simulink model "ChoiSul1996_DeadTime"  (R2024b)
settings: Solver=FixedStepDiscrete  StartTime=0.0  StopTime=Duration  FixedStep=h  RelTol=1e-3
InitFcn:
  | demoModel=bdroot; demoWorkspace=get_param(demoModel,'ModelWorkspace');
  | demoCases=getVariable(demoWorkspace,'DemoCases');
  | demoCaseName=get_param([demoModel '/Experiment_Settings'],'CaseName');
  | demoSelected=find(strcmp(demoCaseName,{demoCases.name}),1);
  | demoValues=demoCases(demoSelected).variables; demoNames=fieldnames(demoValues);
  | for demoIndex=1:numel(demoNames), assignin(demoWorkspace,demoNames{demoIndex},demoValues.(demoNames{demoIndex})); end
  | clear demoModel demoWorkspace demoCases demoCaseName demoSelected demoValues demoNames demoIndex;
model workspace (MAT data in the model file):
  CompDuty = 0.0266762524843
  DemoCases(1).name = 'No_compensation'
  DemoCases(1).variables.CompDuty = 0
  DemoCases(1).variables.UseWeakening = 0
  DemoCases(2).name = 'Calibrated_compensation'
  DemoCases(2).variables.CompDuty = 0.0266762524843
  DemoCases(2).variables.UseWeakening = 0
  SpeedProgram = [0  0; 0.12  300; 0.9  300]
  UseWeakening = 0
values from neighbouring files (symbols this model uses):
  B = 0.0002    [ChoiSul1996_DeadTime.sldd]
  BaseCap = 11.4197598 11.4197598 11.4197598 11.4197598 11.4197598 11.4197598 11.4197598 11.4197598 11.4197598 11.4197598 11.4197598 11.4197598 11.4197598 11.4197598 11.4197598 11.4197598 11.4197598 11.4197598 11.4197598 11.4197598 11.4197598 11.4197598 11.4197598 11.4197598 11.4197598 11.4197598 11.4197598 11.4197598 11.4197598 11.4197598 11.4197598 11.4197598 11.4197598 11.4197598 11.4197598 11.4197598 11.4    [ChoiSul1996_DeadTime.sldd]
  BaseId = -0.0 -0.0 -0.0 -0.0 -0.0 -0.0 -0.0 -0.0 -0.0 -0.0 -0.0 -0.0 -0.0 -0.0 -0.0 -0.0 -0.0 -0.0 -0.0 -0.0 -0.0 -0.0 -0.0 -0.0 -0.0 -0.0 -0.0 -0.0 -0.0 -0.0 -0.0 -0.0 -0.0 -0.0 -0.0 -0.0 -0.0 -0.0 -0.0 -0.0 -0.0 -0.0 -0.0 -0.0 -0.0 -0.0 -0.0 -0.0 -0.0 -0.0 -0.0 -0.0 -0.0 -0.0 -0.0 -0.0 -0.0 -0.0 -0.0 -0.0 -0.0 -0.0 -0.0 -0.0 -0.0 -0.0 -0.0 -0.0 -0.0 -0.0 -0.0 -0.0 -0.0 -0.0 -0.0 -0.0 -0.0 -0.0 -0.0 -0.0    [ChoiSul1996_DeadTime.sldd]
  BaseIq = 0.0 0.0 0.0 0.0 0.0 0.0 0.0 0.0 0.0 0.0 0.0 0.0 0.0 0.0 0.0 0.0 0.0 0.0 0.0 0.0 0.0 0.0 0.0 0.0 0.0 0.0 0.0 0.0 0.0 0.0 0.0 0.0 0.0 0.0 0.0 0.0 0.0 0.0 0.0 0.0 0.0 0.0 0.0 0.0 0.0 0.0 0.0 0.0 0.0 0.0 0.0 0.0 0.0 0.0 0.0 0.0 0.0 0.0 0.0 0.0 0.0 0.0 0.0 0.0 0.0 0.0 0.0 0.0 0.0 0.0 0.0 0.0 0.0 0.0 0.0 0.0 0.0 0.0 0.0 0.0 0.0 0.0 0.0 0.0 0.0 0.0 0.0 0.0 0.0 0.0 0.0 0.0 0.0 0.0 0.0 0.0 0.0 0.0 0.0 0.0    [ChoiSul1996_DeadTime.sldd]
  BusReadyRatio = 0.94    [ChoiSul1996_DeadTime.sldd]
  CurrentBandwidth = 1450.0    [ChoiSul1996_DeadTime.sldd]
  CurrentKaw = 1500.0    [ChoiSul1996_DeadTime.sldd]
  EdgePredict = 0.27    [ChoiSul1996_DeadTime.sldd]
  EnableThreshold = 0.5    [ChoiSul1996_DeadTime.sldd]
  Fraction = 0.0 0.025 0.05 0.075 0.1 0.125 0.15 0.175 0.2 0.225 0.25 0.275 0.3 0.325 0.35 0.375 0.4 0.425 0.45 0.475 0.5 0.525 0.55 0.575 0.6 0.625 0.65 0.675 0.7 0.725 0.75 0.775 0.8 0.825 0.85 0.875 0.9 0.925 0.95 0.975 1.0    [ChoiSul1996_DeadTime.sldd]
  FwCap = 11.4197598 11.4197598 11.4197598 11.4197598 11.4197598 11.4197598 11.4197598 11.4197598 11.4197598 11.4197598 11.4197598 11.4197598 11.4197598 11.4197598 11.4197598 11.4197598 11.4197598 11.4197598 11.4197598 11.4197598 11.4197598 11.4197598 11.4197598 11.4197598 11.4197598 11.4197598 11.4197598 11.4197598 11.4197598 11.4197598 11.4197598 11.4197598 11.4197598 11.4197598 11.4197598 11.4197598 11.4    [ChoiSul1996_DeadTime.sldd]
  FwId = -0.0 -0.0 -0.0 -0.0 -0.0 -0.0 -0.0 -0.0 -0.0 -0.0 -0.0 -0.0 -0.0 -0.0 -0.0 -0.0 -0.0 -0.0 -0.0 -0.0 -0.0 -0.0 -0.0 -0.0 -0.0 -0.0 -0.0 -0.0 -0.0 -0.0 -0.0 -0.0 -0.0 -0.0 -0.0 -0.0 -0.0 -0.0 -0.0 -0.0 -0.0 -0.0 -0.0 -0.0 -0.0 -0.0 -0.0 -0.0 -0.0 -0.0 -0.0 -0.0 -0.0 -0.0 -0.0 -0.0 -0.0 -0.0 -0.0 -0.0 -0.0 -0.0 -0.0 -0.0 -0.0 -0.0 -0.0 -0.0 -0.0 -0.0 -0.0 -0.0 -0.0 -0.0 -0.0 -0.0 -0.0 -0.0 -0.0 -0.0    [ChoiSul1996_DeadTime.sldd]
  FwIq = 0.0 0.0 0.0 0.0 0.0 0.0 0.0 0.0 0.0 0.0 0.0 0.0 0.0 0.0 0.0 0.0 0.0 0.0 0.0 0.0 0.0 0.0 0.0 0.0 0.0 0.0 0.0 0.0 0.0 0.0 0.0 0.0 0.0 0.0 0.0 0.0 0.0 0.0 0.0 0.0 0.0 0.0 0.0 0.0 0.0 0.0 0.0 0.0 0.0 0.0 0.0 0.0 0.0 0.0 0.0 0.0 0.0 0.0 0.0 0.0 0.0 0.0 0.0 0.0 0.0 0.0 0.0 0.0 0.0 0.0 0.0 0.0 0.0 0.0 0.0 0.0 0.0 0.0 0.0 0.0 0.0 0.0 0.0 0.0 0.0 0.0 0.0 0.0 0.0 0.0 0.0 0.0 0.0 0.0 0.0 0.0 0.0 0.0 0.0 0.0    [ChoiSul1996_DeadTime.sldd]
  h = 1.0E-6    [ChoiSul1996_DeadTime.sldd]
  J = 0.0006    [ChoiSul1996_DeadTime.sldd]
  Ld = 0.001875    [ChoiSul1996_DeadTime.sldd]
  Lq = 0.00375    [ChoiSul1996_DeadTime.sldd]
  NearZeroInvA = 4.347826    [ChoiSul1996_DeadTime.sldd]
  Ngrid = 0.0 25.0 50.0 75.0 100.0 125.0 150.0 175.0 200.0 225.0 250.0 275.0 300.0 325.0 350.0 375.0 400.0 425.0 450.0 475.0 500.0 525.0 550.0 575.0 600.0 625.0 650.0 675.0 700.0 725.0 750.0 775.0 800.0 825.0 850.0 875.0 900.0 925.0 950.0 975.0 1000.0 1025.0 1050.0 1075.0 1100.0 1125.0 1150.0 1175.0 1200.0 1225.0 1250.0 1275.0 1300.0 1325.0 1350.0 1375.0 1400.0 1425.0 1450.0 1475.0 1500.0 1525.0 1550.0 1575    [ChoiSul1996_DeadTime.sldd]
  Pairs = 4.0    [ChoiSul1996_DeadTime.sldd]
  Psi = 0.045    [ChoiSul1996_DeadTime.sldd]
  R = 0.065    [ChoiSul1996_DeadTime.sldd]
  SpeedKaw = 90.0    [ChoiSul1996_DeadTime.sldd]
  SpeedKi = 1.3    [ChoiSul1996_DeadTime.sldd]
  SpeedKp = 0.018    [ChoiSul1996_DeadTime.sldd]
  Ts = 0.0001    [ChoiSul1996_DeadTime.sldd]
  Vdc = 86.602540378443862    [ChoiSul1996_DeadTime.sldd]
  VoltageUtilization = 0.98    [ChoiSul1996_DeadTime.sldd]
(part 1 of 2)
settings Model: DataDictionary=ChoiSul1996_DeadTime.sldd  Creator=lxy  LastModifiedBy=lxy
settings DataIOCC: SaveOutput=off  SaveTime=off

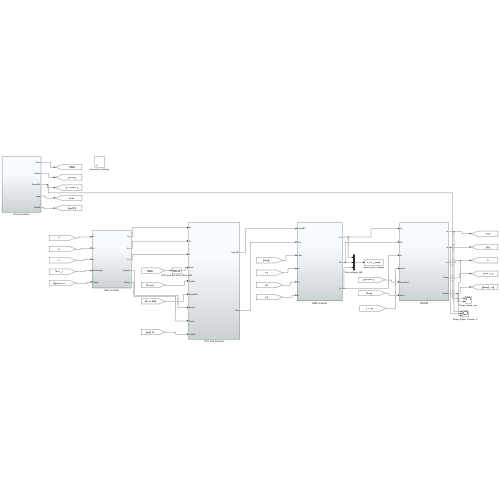
[thumbnail: Simulink's stored preview of the top-level diagram]
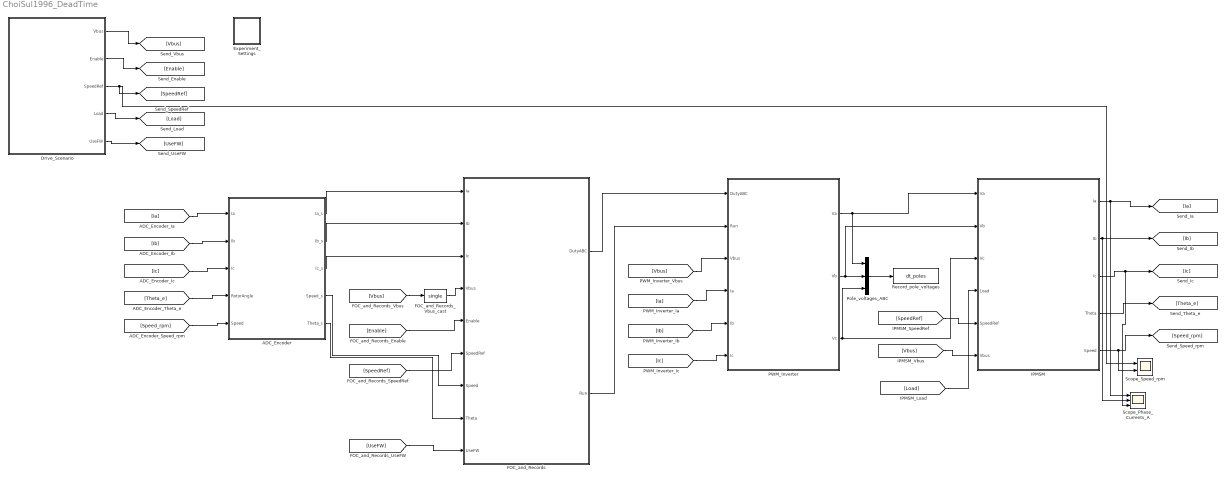
== system ChoiSul1996_DeadTime ==
  ADC_Encoder : Subsystem
  Drive_Scenario : Subsystem
  Experiment_Settings : Subsystem  mask{CaseName=Calibrated_compensation}
      mask prompts: CaseName "Experiment"
      mask help: Select the experiment, then click Run. Parameters and test inputs are included in the download.
      mask TypeOptions CaseName: No_compensation | Calibrated_compensation
  FOC_and_Records : Subsystem
  FOC_and_Records_Vbus_cast : DataTypeConversion  OutDataTypeStr=single  SaturateOnIntegerOverflow=off  RndMeth=Floor
  IPMSM : Subsystem
  PWM_Inverter : Subsystem
  Pole_voltages_ABC : Mux  Inputs=3
  Record_pole_voltages : ToWorkspace  VariableName=dt_poles  SaveFormat=Timeseries  SampleTime=-1
  Scope_Phase_Currents_A : Scope  NumInputPorts=3
  Scope_Speed_rpm : Scope  NumInputPorts=2
  wires:
  [Vbus] -> IPMSM/6(Vbus)
  [SpeedRef] -> IPMSM/5(SpeedRef)
  [Ic] -> PWM_Inverter/6(Ic)
  [Ib] -> PWM_Inverter/5(Ib)
  [Ia] -> PWM_Inverter/4(Ia)
  [Vbus] -> PWM_Inverter/3(Vbus)
  FOC_and_Records/2(Run) -> PWM_Inverter/2(Run)
  FOC_and_Records/1(DutyABC) -> PWM_Inverter/1(DutyABC)
  [UseFW] -> FOC_and_Records/9(UseFW)
  [SpeedRef] -> FOC_and_Records/6(SpeedRef)
  [Enable] -> FOC_and_Records/5(Enable)
  FOC_and_Records_Vbus_cast/1 -> FOC_and_Records/4(Vbus)
  [Vbus] -> FOC_and_Records_Vbus_cast/1
  ADC_Encoder/5(Theta_s) -> FOC_and_Records/8(Theta)
  ADC_Encoder/4(Speed_s) -> FOC_and_Records/7(Speed)
  ADC_Encoder/3(Ic_s) -> FOC_and_Records/3(Ic)
  ADC_Encoder/2(Ib_s) -> FOC_and_Records/2(Ib)
  ADC_Encoder/1(Ia_s) -> FOC_and_Records/1(Ia)
  [Speed_rpm] -> ADC_Encoder/5(Speed)
  [Theta_e] -> ADC_Encoder/4(RotorAngle)
  [Ic] -> ADC_Encoder/3(Ic)
  [Ib] -> ADC_Encoder/2(Ib)
  [Ia] -> ADC_Encoder/1(Ia)
  IPMSM/4(Theta) -> [Theta_e]
  IPMSM/3(Ic) -> Scope_Phase_Currents_A/3, [Ic]
  Drive_Scenario/5(UseFW) -> [UseFW]
  Drive_Scenario/4(Load) -> [Load]
  Drive_Scenario/2(Enable) -> [Enable]
  Drive_Scenario/1(Vbus) -> [Vbus]
  Pole_voltages_ABC/1 -> Record_pole_voltages/1
  PWM_Inverter/1(Va) -> Pole_voltages_ABC/1, IPMSM/1(Va)
  PWM_Inverter/2(Vb) -> IPMSM/2(Vb), Pole_voltages_ABC/2
  PWM_Inverter/3(Vc) -> IPMSM/3(Vc), Pole_voltages_ABC/3
  [Load] -> IPMSM/4(Load)
  Drive_Scenario/3(SpeedRef) -> Scope_Speed_rpm/1, [SpeedRef]
  IPMSM/5(Speed) -> Scope_Speed_rpm/2, [Speed_rpm]
  IPMSM/1(Ia) -> [Ia], Scope_Phase_Currents_A/1
  IPMSM/2(Ib) -> Scope_Phase_Currents_A/2, [Ib]

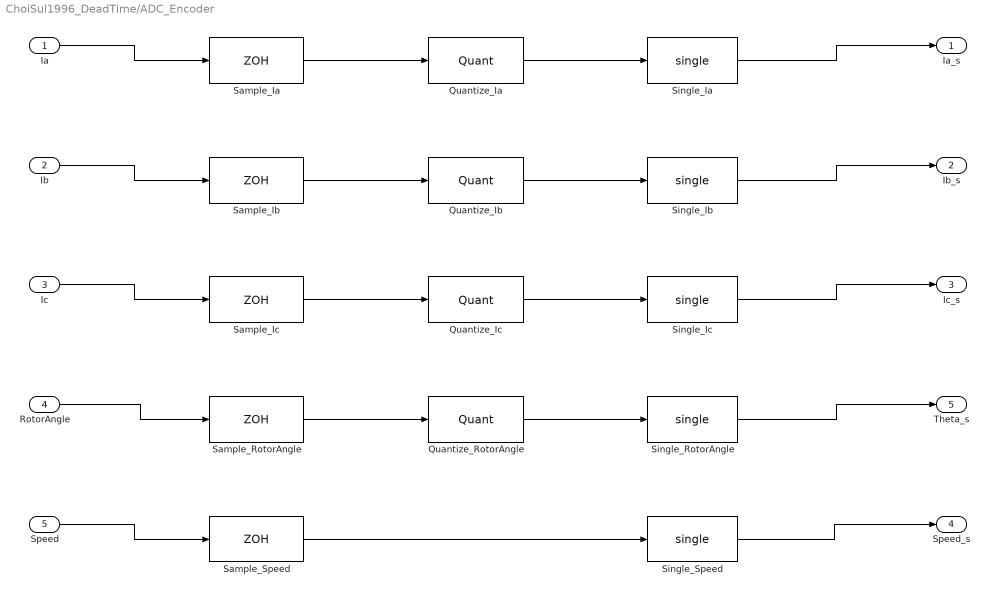
== system ChoiSul1996_DeadTime/ADC_Encoder ==
  Ia : Inport
  Ib : Inport  Port=2
  Ic : Inport  Port=3
  RotorAngle : Inport  Port=4
  Speed : Inport  Port=5
  Quantize_Ia : Quantizer  QuantizationInterval=0.02
  Quantize_Ib : Quantizer  QuantizationInterval=0.02
  Quantize_Ic : Quantizer  QuantizationInterval=0.02
  Quantize_RotorAngle : Quantizer  QuantizationInterval=2*pi*Pairs/16384
  Sample_Ia : ZeroOrderHold  SampleTime=Ts
  Sample_Ib : ZeroOrderHold  SampleTime=Ts
  Sample_Ic : ZeroOrderHold  SampleTime=Ts
  Sample_RotorAngle : ZeroOrderHold  SampleTime=Ts
  Sample_Speed : ZeroOrderHold  SampleTime=Ts
  Single_Ia : DataTypeConversion  OutDataTypeStr=single  SaturateOnIntegerOverflow=off  RndMeth=Floor
  Single_Ib : DataTypeConversion  OutDataTypeStr=single  SaturateOnIntegerOverflow=off  RndMeth=Floor
  Single_Ic : DataTypeConversion  OutDataTypeStr=single  SaturateOnIntegerOverflow=off  RndMeth=Floor
  Single_RotorAngle : DataTypeConversion  OutDataTypeStr=single  SaturateOnIntegerOverflow=off  RndMeth=Floor
  Single_Speed : DataTypeConversion  OutDataTypeStr=single  SaturateOnIntegerOverflow=off  RndMeth=Floor
  Ia_s : Outport
  Ib_s : Outport  Port=2
  Ic_s : Outport  Port=3
  Speed_s : Outport  Port=4
  Theta_s : Outport  Port=5
  wires:
  Single_Ib/1 -> Ib_s/1
  Single_RotorAngle/1 -> Theta_s/1
  Single_Ic/1 -> Ic_s/1
  Single_Ia/1 -> Ia_s/1
  Quantize_Ib/1 -> Single_Ib/1
  Quantize_RotorAngle/1 -> Single_RotorAngle/1
  Quantize_Ic/1 -> Single_Ic/1
  Quantize_Ia/1 -> Single_Ia/1
  Single_Speed/1 -> Speed_s/1
  Sample_RotorAngle/1 -> Quantize_RotorAngle/1
  Sample_Speed/1 -> Single_Speed/1
  Ib/1 -> Sample_Ib/1
  Sample_Ia/1 -> Quantize_Ia/1
  RotorAngle/1 -> Sample_RotorAngle/1
  Sample_Ic/1 -> Quantize_Ic/1
  Ic/1 -> Sample_Ic/1
  Speed/1 -> Sample_Speed/1
  Ia/1 -> Sample_Ia/1
  Sample_Ib/1 -> Quantize_Ib/1

== system ChoiSul1996_DeadTime/Drive_Scenario ==
  DC_bus : Constant  Value=Vdc  OutDataTypeStr=double  SampleTime=Ts
  Enable_drive : Step  Time=0.015  SampleTime=Ts
  Enable_single : DataTypeConversion  OutDataTypeStr=single  SaturateOnIntegerOverflow=off  RndMeth=Floor
  Load_torque : Step  Time=1.18  Before=0.70  After=1.30  SampleTime=h
  Reference_single : DataTypeConversion  OutDataTypeStr=single  SaturateOnIntegerOverflow=off  RndMeth=Floor
  Speed_program : FromWorkspace  VariableName=SpeedProgram  SampleTime=Ts
  Strategy : Constant  Value=UseWeakening  OutDataTypeStr=single  SampleTime=Ts
  Vbus : Outport
  Enable : Outport  Port=2
  SpeedRef : Outport  Port=3
  Load : Outport  Port=4
  UseFW : Outport  Port=5
  wires:
  Reference_single/1 -> SpeedRef/1
  Enable_drive/1 -> Enable_single/1
  Strategy/1 -> UseFW/1
  Load_torque/1 -> Load/1
  DC_bus/1 -> Vbus/1
  Speed_program/1 -> Reference_single/1
  Enable_single/1 -> Enable/1

== system ChoiSul1996_DeadTime/Experiment_Settings ==

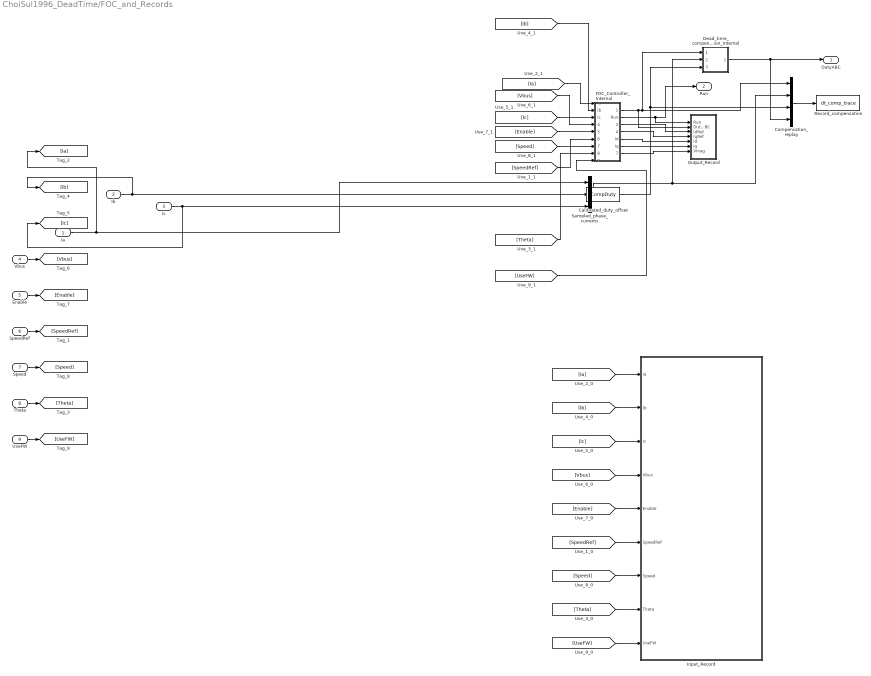
== system ChoiSul1996_DeadTime/FOC_and_Records ==
  Ia : Inport
  Ib : Inport  Port=2
  Ic : Inport  Port=3
  Vbus : Inport  Port=4
  Enable : Inport  Port=5
  SpeedRef : Inport  Port=6
  Speed : Inport  Port=7
  Theta : Inport  Port=8
  UseFW : Inport  Port=9
  Calibrated_duty_offset : Constant  Value=CompDuty  OutDataTypeStr=single  SampleTime=Ts
  Compensation_replay : Mux
  Dead_time_compensation_Internal : Subsystem  TreatAsAtomicUnit=on
  FOC_Controller_Internal : Subsystem  TreatAsAtomicUnit=on
  Input_Record : Subsystem
  Output_Record : Subsystem
  Record_compensation : ToWorkspace  VariableName=dt_comp_trace  SaveFormat=Timeseries  SampleTime=-1
  Sampled_phase_currents : Mux  Inputs=3
  DutyABC : Outport
  Run : Outport  Port=2
  wires:
  UseFW/1 -> [UseFW]
  Speed/1 -> [Speed]
  Enable/1 -> [Enable]
  Vbus/1 -> [Vbus]
  Theta/1 -> [Theta]
  SpeedRef/1 -> [SpeedRef]
  [UseFW] -> Input_Record/9(UseFW)
  [Speed] -> Input_Record/7(Speed)
  [Enable] -> Input_Record/5(Enable)
  [Vbus] -> Input_Record/4(Vbus)
  [Ic] -> Input_Record/3(Ic)
  [Ib] -> Input_Record/2(Ib)
  [Theta] -> Input_Record/8(Theta)
  [Ia] -> Input_Record/1(Ia)
  [SpeedRef] -> Input_Record/6(SpeedRef)
  FOC_Controller_Internal/7(Vmag) -> Output_Record/7(Vmag)
  FOC_Controller_Internal/6(Iq) -> Output_Record/6(Iq)
  FOC_Controller_Internal/5(Id) -> Output_Record/5(Id)
  FOC_Controller_Internal/4(IqRef) -> Output_Record/4(IqRef)
  FOC_Controller_Internal/3(IdRef) -> Output_Record/3(IdRef)
  FOC_Controller_Internal/2(Run) -> Run/1, Output_Record/1(Run)
  FOC_Controller_Internal/1(DutyABC) -> Dead_time_compensation_Internal/1(DutyABC), Compensation_replay/1, Output_Record/2(DutyABC)
  [UseFW] -> FOC_Controller_Internal/9(UseFW)
  [Theta] -> FOC_Controller_Internal/8(Theta)
  [Speed] -> FOC_Controller_Internal/7(Speed)
  [SpeedRef] -> FOC_Controller_Internal/6(SpeedRef)
  [Enable] -> FOC_Controller_Internal/5(Enable)
  [Vbus] -> FOC_Controller_Internal/4(Vbus)
  [Ic] -> FOC_Controller_Internal/3(Ic)
  [Ib] -> FOC_Controller_Internal/2(Ib)
  [Ia] -> FOC_Controller_Internal/1(Ia)
  Compensation_replay/1 -> Record_compensation/1
  Calibrated_duty_offset/1 -> Compensation_replay/3, Dead_time_compensation_Internal/3(CompDuty)
  Sampled_phase_currents/1 -> Compensation_replay/2, Dead_time_compensation_Internal/2(CurrentABC_A)
  Ia/1 -> Sampled_phase_currents/1, [Ia]
  Ib/1 -> Sampled_phase_currents/2, [Ib]
  Ic/1 -> Sampled_phase_currents/3, [Ic]
  Dead_time_compensation_Internal/1(DutyCorrectedABC) -> Compensation_replay/4, DutyABC/1

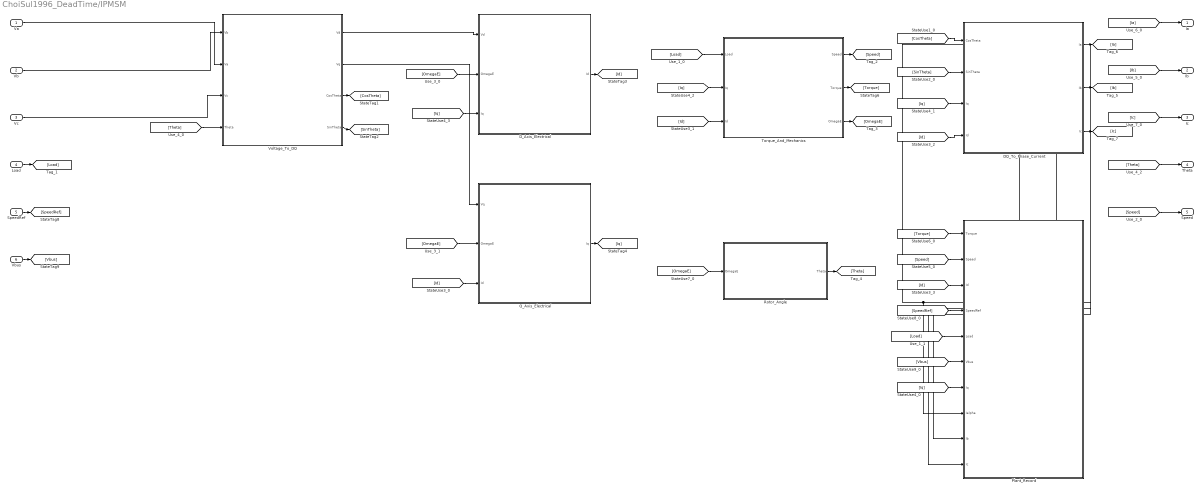
== system ChoiSul1996_DeadTime/IPMSM ==
  Va : Inport
  Vb : Inport  Port=2
  Vc : Inport  Port=3
  Load : Inport  Port=4
  SpeedRef : Inport  Port=5
  Vbus : Inport  Port=6
  DQ_To_Phase_Current : Subsystem
  D_Axis_Electrical : Subsystem
  Plant_Record : Subsystem
  Q_Axis_Electrical : Subsystem
  Rotor_Angle : Subsystem
  Torque_And_Mechanics : Subsystem
  Voltage_To_DQ : Subsystem
  Ia : Outport
  Ib : Outport  Port=2
  Ic : Outport  Port=3
  Theta : Outport  Port=4
  Speed : Outport  Port=5
  wires:
  Load/1 -> [Load]
  [Ic] -> Ic/1
  [Ia] -> Ia/1
  [Ib] -> Ib/1
  [Theta] -> Theta/1
  [Speed] -> Speed/1
  [Load] -> Torque_And_Mechanics/1(Load)
  Torque_And_Mechanics/1(Speed) -> [Speed]
  Torque_And_Mechanics/3(OmegaE) -> [OmegaE]
  [Vbus] -> Plant_Record/6(Vbus)
  [SpeedRef] -> Plant_Record/4(SpeedRef)
  [OmegaE] -> Rotor_Angle/1(OmegaE)
  [Torque] -> Plant_Record/1(Torque)
  [Speed] -> Plant_Record/2(Speed)
  [Iq] -> D_Axis_Electrical/3(Iq)
  [Iq] -> Torque_And_Mechanics/2(Iq)
  [Iq] -> DQ_To_Phase_Current/3(Iq)
  [Iq] -> Plant_Record/7(Iq)
  [Id] -> Plant_Record/3(Id)
  [Id] -> DQ_To_Phase_Current/4(Id)
  [Id] -> Torque_And_Mechanics/3(Id)
  [Id] -> Q_Axis_Electrical/3(Id)
  [SinTheta] -> DQ_To_Phase_Current/2(SinTheta)
  [CosTheta] -> DQ_To_Phase_Current/1(CosTheta)
  Voltage_To_DQ/4(SinTheta) -> [SinTheta]
  Voltage_To_DQ/3(CosTheta) -> [CosTheta]
  DQ_To_Phase_Current/3(Ic) -> Plant_Record/10(Ic), [Ic]
  DQ_To_Phase_Current/1(Ia) -> [Ia], Plant_Record/8(Ialpha)
  DQ_To_Phase_Current/2(Ib) -> Plant_Record/9(Ib), [Ib]
  Rotor_Angle/1(Theta) -> [Theta]
  Torque_And_Mechanics/2(Torque) -> [Torque]
  Voltage_To_DQ/2(Vq) -> Q_Axis_Electrical/1(Vq)
  Q_Axis_Electrical/1(Iq) -> [Iq]
  Voltage_To_DQ/1(Vd) -> D_Axis_Electrical/1(Vd)
  D_Axis_Electrical/1(Id) -> [Id]
  [Load] -> Plant_Record/5(Load)
  [OmegaE] -> D_Axis_Electrical/2(OmegaE)
  [OmegaE] -> Q_Axis_Electrical/2(OmegaE)
  [Theta] -> Voltage_To_DQ/4(Theta)
  SpeedRef/1 -> [SpeedRef]
  Vbus/1 -> [Vbus]
  Vb/1 -> Voltage_To_DQ/1(Vb)
  Va/1 -> Voltage_To_DQ/2(Va)
  Vc/1 -> Voltage_To_DQ/3(Vc)

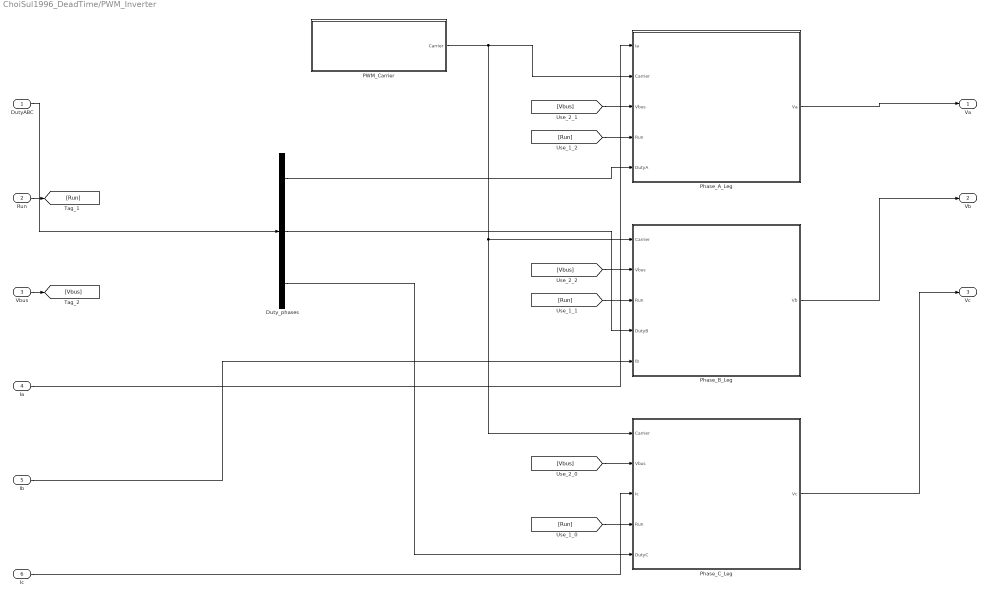
== system ChoiSul1996_DeadTime/PWM_Inverter ==
  DutyABC : Inport
  Run : Inport  Port=2
  Vbus : Inport  Port=3
  Ia : Inport  Port=4
  Ib : Inport  Port=5
  Ic : Inport  Port=6
  Duty_phases : Demux  Outputs=3
  PWM_Carrier : Subsystem
  Phase_A_Leg : Subsystem
  Phase_B_Leg : Subsystem
  Phase_C_Leg : Subsystem
  Va : Outport
  Vb : Outport  Port=2
  Vc : Outport  Port=3
  wires:
  Phase_C_Leg/1(Vc) -> Vc/1
  Ic/1 -> Phase_C_Leg/3(Ic)
  Phase_B_Leg/1(Vb) -> Vb/1
  Ib/1 -> Phase_B_Leg/5(Ib)
  Phase_A_Leg/1(Va) -> Va/1
  Ia/1 -> Phase_A_Leg/1(Ia)
  PWM_Carrier/1(Carrier) -> Phase_C_Leg/1(Carrier), Phase_B_Leg/1(Carrier), Phase_A_Leg/2(Carrier)
  Vbus/1 -> [Vbus]
  Run/1 -> [Run]
  DutyABC/1 -> Duty_phases/1
  [Vbus] -> Phase_B_Leg/2(Vbus)
  [Vbus] -> Phase_A_Leg/3(Vbus)
  [Vbus] -> Phase_C_Leg/2(Vbus)
  [Run] -> Phase_A_Leg/4(Run)
  [Run] -> Phase_B_Leg/3(Run)
  [Run] -> Phase_C_Leg/4(Run)
  Duty_phases/1 -> Phase_A_Leg/5(DutyA)
  Duty_phases/2 -> Phase_B_Leg/4(DutyB)
  Duty_phases/3 -> Phase_C_Leg/5(DutyC)

== system ChoiSul1996_DeadTime/FOC_and_Records/Dead_time_compensation_Internal ==
  DutyABC : Inport  OutDataTypeStr=single  PortDimensions=3  SampleTime=Ts
  CurrentABC_A : Inport  Port=2  OutDataTypeStr=single  PortDimensions=3  SampleTime=Ts
  CompDuty : Inport  Port=3  OutDataTypeStr=single  PortDimensions=1  SampleTime=Ts
  Calibrated_correction : Product  Inputs=**
  Corrected_command : Sum
  Current_change : Sum  Inputs=+-
  Estimated_edge_current : Sum
  Keep_pulse_headroom : Saturate  UpperLimit=0.97  LowerLimit=0.03
  Normalize_near_zero : Gain  Gain=NearZeroInvA
  Predict_to_edge : Gain  Gain=EdgePredict
  Previous_current : UnitDelay  SampleTime=Ts  HasFrameUpgradeWarning=on
  Smooth_polarity : Saturate  UpperLimit=1  LowerLimit=-1
  DutyCorrectedABC : Outport
  wires:
  Keep_pulse_headroom/1 -> DutyCorrectedABC/1
  Corrected_command/1 -> Keep_pulse_headroom/1
  Calibrated_correction/1 -> Corrected_command/2
  DutyABC/1 -> Corrected_command/1
  CompDuty/1 -> Calibrated_correction/2
  Smooth_polarity/1 -> Calibrated_correction/1
  Normalize_near_zero/1 -> Smooth_polarity/1
  Estimated_edge_current/1 -> Normalize_near_zero/1
  Predict_to_edge/1 -> Estimated_edge_current/2
  Current_change/1 -> Predict_to_edge/1
  Previous_current/1 -> Current_change/2
  CurrentABC_A/1 -> Estimated_edge_current/1, Current_change/1, Previous_current/1

== system ChoiSul1996_DeadTime/FOC_and_Records/FOC_Controller_Internal ==
  Ia : Inport  Description=A；A相瞬时电流；single；100 us  OutDataTypeStr=single  SampleTime=Ts
  Ib : Inport  Description=A；B相瞬时电流；single；100 us  Port=2  OutDataTypeStr=single  SampleTime=Ts
  Ic : Inport  Description=A；C相瞬时电流；single；100 us  Port=3  OutDataTypeStr=single  SampleTime=Ts
  Vbus : Inport  Description=V；同步测得的直流母线；single  Port=4  OutDataTypeStr=single  SampleTime=Ts
  Enable : Inport  Description=0或1；运行请求；single；失能时下一周期清零PI状态  Port=5  OutDataTypeStr=single  SampleTime=Ts
  SpeedRef : Inport  Description=机械转速指令，rpm；single  Port=6  OutDataTypeStr=single  SampleTime=Ts
  Speed : Inport  Description=机械转速反馈，rpm；single  Port=7  OutDataTypeStr=single  SampleTime=Ts
  Theta : Inport  Description=电角度，rad；按A-B-C相序标定；single  Port=8  OutDataTypeStr=single  SampleTime=Ts
  UseFW : Inport  Description=0=常规MTPA，1=电压电流约束下弱磁；single  Port=9  OutDataTypeStr=single  SampleTime=Ts
  FOC_Model : Subsystem  Description=可独立移植的FOC控制器。100 us固定离散执行；依赖同目录morimoto_params.sldd。速度环、两轴电流环、MTPA/弱磁查表、解耦及SVPWM均由原生模块展开。  TreatAsAtomicUnit=on
  DutyABC : Outport  Description=三相归一化占空比[0,1]；3个single；板级适配层换算定时器计数
  Run : Outport  Description=运行联锁boolean；为0时硬件关闭PWM输出  Port=2
  IdRef : Outport  Description=d轴电流指令，A；single  Port=3
  IqRef : Outport  Description=q轴电流指令，A；single  Port=4
  Id : Outport  Description=采样变换后的d轴电流，A  Port=5
  Iq : Outport  Description=采样变换后的q轴电流，A  Port=6
  Vmag : Outport  Description=限幅后的电压矢量幅值，V  Port=7
  wires:
  Ia/1 -> FOC_Model/1(Ia)
  Ib/1 -> FOC_Model/2(Ib)
  Ic/1 -> FOC_Model/3(Ic)
  Vbus/1 -> FOC_Model/4(Vbus)
  Enable/1 -> FOC_Model/5(Enable)
  SpeedRef/1 -> FOC_Model/6(SpeedRef)
  Speed/1 -> FOC_Model/7(Speed)
  Theta/1 -> FOC_Model/8(Theta)
  UseFW/1 -> FOC_Model/9(UseFW)
  FOC_Model/1(DutyABC) -> DutyABC/1
  FOC_Model/3(IdRef) -> IdRef/1
  FOC_Model/4(IqRef) -> IqRef/1
  FOC_Model/5(Id) -> Id/1
  FOC_Model/6(Iq) -> Iq/1
  FOC_Model/7(Vmag) -> Vmag/1
  FOC_Model/2(Run) -> Run/1

== system ChoiSul1996_DeadTime/FOC_and_Records/Input_Record ==
  Ia : Inport
  Ib : Inport  Port=2
  Ic : Inport  Port=3
  Vbus : Inport  Port=4
  Enable : Inport  Port=5
  SpeedRef : Inport  Port=6
  Speed : Inport  Port=7
  Theta : Inport  Port=8
  UseFW : Inport  Port=9
  sampled_inputs : ToWorkspace  VariableName=sampled_inputs  SaveFormat=Timeseries  SampleTime=-1
  sampled_inputs_bus : Mux  Inputs=9
  sampled_inputs_value_{1..9} (9 alike) : DataTypeConversion  OutDataTypeStr=double  SaturateOnIntegerOverflow=off  RndMeth=Floor
  wires:
  Ic/1 -> sampled_inputs_value_3/1
  Ib/1 -> sampled_inputs_value_2/1
  UseFW/1 -> sampled_inputs_value_9/1
  Enable/1 -> sampled_inputs_value_5/1
  SpeedRef/1 -> sampled_inputs_value_6/1
  Vbus/1 -> sampled_inputs_value_4/1
  Theta/1 -> sampled_inputs_value_8/1
  Ia/1 -> sampled_inputs_value_1/1
  sampled_inputs_value_8/1 -> sampled_inputs_bus/8
  sampled_inputs_value_4/1 -> sampled_inputs_bus/4
  sampled_inputs_value_9/1 -> sampled_inputs_bus/9
  Speed/1 -> sampled_inputs_value_7/1
  sampled_inputs_value_7/1 -> sampled_inputs_bus/7
  sampled_inputs_bus/1 -> sampled_inputs/1
  sampled_inputs_value_5/1 -> sampled_inputs_bus/5
  sampled_inputs_value_6/1 -> sampled_inputs_bus/6
  sampled_inputs_value_2/1 -> sampled_inputs_bus/2
  sampled_inputs_value_3/1 -> sampled_inputs_bus/3
  sampled_inputs_value_1/1 -> sampled_inputs_bus/1

== system ChoiSul1996_DeadTime/FOC_and_Records/Output_Record ==
  Run : Inport
  DutyABC : Inport  Port=2
  IdRef : Inport  Port=3
  IqRef : Inport  Port=4
  Id : Inport  Port=5
  Iq : Inport  Port=6
  Vmag : Inport  Port=7
  sampled_outputs : ToWorkspace  VariableName=sampled_outputs  SaveFormat=Timeseries  SampleTime=-1
  sampled_outputs_bus : Mux  Inputs=7
  sampled_outputs_value_{1..7} (7 alike) : DataTypeConversion  OutDataTypeStr=double  SaturateOnIntegerOverflow=off  RndMeth=Floor
  wires:
  Id/1 -> sampled_outputs_value_5/1
  IqRef/1 -> sampled_outputs_value_4/1
  DutyABC/1 -> sampled_outputs_value_1/1
  Run/1 -> sampled_outputs_value_2/1
  Iq/1 -> sampled_outputs_value_6/1
  sampled_outputs_value_1/1 -> sampled_outputs_bus/1
  sampled_outputs_value_2/1 -> sampled_outputs_bus/2
  sampled_outputs_value_6/1 -> sampled_outputs_bus/6
  IdRef/1 -> sampled_outputs_value_3/1
  sampled_outputs_value_5/1 -> sampled_outputs_bus/5
  sampled_outputs_bus/1 -> sampled_outputs/1
  sampled_outputs_value_3/1 -> sampled_outputs_bus/3
  Vmag/1 -> sampled_outputs_value_7/1
  sampled_outputs_value_7/1 -> sampled_outputs_bus/7
  sampled_outputs_value_4/1 -> sampled_outputs_bus/4

== system ChoiSul1996_DeadTime/IPMSM/DQ_To_Phase_Current ==
  CosTheta : Inport
  SinTheta : Inport  Port=2
  Iq : Inport  Port=3
  Id : Inport  Port=4
  Beta_sqrt3_2 : Gain  Gain=sqrt(3)/2
  D_cos : Product
  D_sin : Product
  Inverse_Alpha : Sum  Inputs=+-
  Inverse_Beta : Sum
  Minus_half_alpha : Gain  Gain=-0.5
  Phase_B : Sum
  Phase_C : Sum  Inputs=+-
  Q_cos : Product
  Q_sin : Product
  Ia : Outport
  Ib : Outport  Port=2
  Ic : Outport  Port=3
  wires:
  Phase_C/1 -> Ic/1
  Phase_B/1 -> Ib/1
  Id/1 -> D_sin/1, D_cos/1
  SinTheta/1 -> Q_sin/2, D_sin/2
  D_cos/1 -> Inverse_Alpha/1
  Beta_sqrt3_2/1 -> Phase_C/2, Phase_B/2
  Q_sin/1 -> Inverse_Alpha/2
  Iq/1 -> Q_sin/1, Q_cos/1
  Inverse_Beta/1 -> Beta_sqrt3_2/1
  Q_cos/1 -> Inverse_Beta/2
  D_sin/1 -> Inverse_Beta/1
  CosTheta/1 -> D_cos/2, Q_cos/2
  Minus_half_alpha/1 -> Phase_B/1, Phase_C/1
  Inverse_Alpha/1 -> Ia/1, Minus_half_alpha/1

== system ChoiSul1996_DeadTime/IPMSM/D_Axis_Electrical ==
  Vd : Inport
  OmegaE : Inport  Port=2
  Iq : Inport  Port=3
  D_current_derivative : Sum  Inputs=+-+
  D_resistive_drop : Gain  Gain=R
  Delta_Id : Gain  Gain=h/Ld
  Id_state : UnitDelay  InitialCondition=double(0)  SampleTime=h  HasFrameUpgradeWarning=on
  Next_Id : Sum
  Q_axis_speed_voltage : Product
  Q_flux : Gain  Gain=Lq
  Id : Outport
  wires:
  Vd/1 -> D_current_derivative/1
  OmegaE/1 -> Q_axis_speed_voltage/1
  Q_flux/1 -> Q_axis_speed_voltage/2
  Iq/1 -> Q_flux/1
  D_current_derivative/1 -> Delta_Id/1
  Q_axis_speed_voltage/1 -> D_current_derivative/3
  Next_Id/1 -> Id_state/1
  Delta_Id/1 -> Next_Id/2
  D_resistive_drop/1 -> D_current_derivative/2
  Id_state/1 -> Next_Id/1, Id/1, D_resistive_drop/1

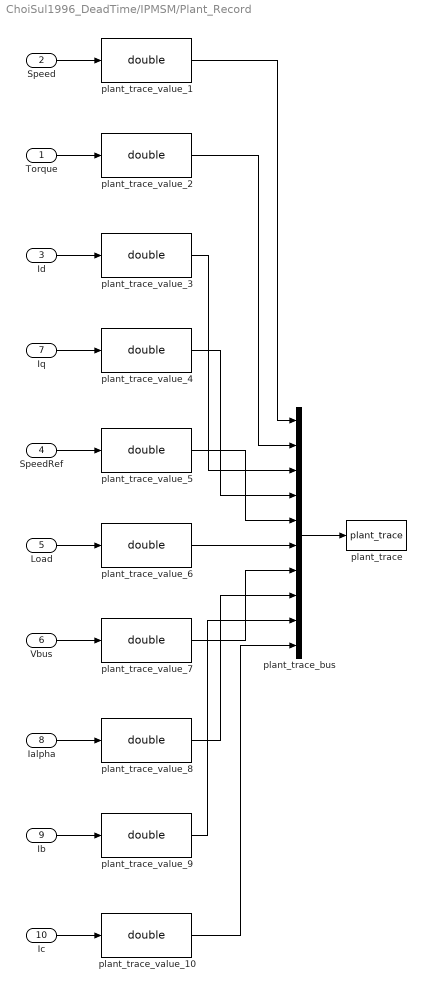
== system ChoiSul1996_DeadTime/IPMSM/Plant_Record ==
  Torque : Inport
  Speed : Inport  Port=2
  Id : Inport  Port=3
  SpeedRef : Inport  Port=4
  Load : Inport  Port=5
  Vbus : Inport  Port=6
  Iq : Inport  Port=7
  Ialpha : Inport  Port=8
  Ib : Inport  Port=9
  Ic : Inport  Port=10
  plant_trace : ToWorkspace  VariableName=plant_trace  SaveFormat=Timeseries  SampleTime=-1
  plant_trace_bus : Mux  Inputs=10
  plant_trace_value_{1..10} (10 alike) : DataTypeConversion  OutDataTypeStr=double  SaturateOnIntegerOverflow=off  RndMeth=Floor
  wires:
  Ic/1 -> plant_trace_value_10/1
  Ialpha/1 -> plant_trace_value_8/1
  Ib/1 -> plant_trace_value_9/1
  SpeedRef/1 -> plant_trace_value_5/1
  Vbus/1 -> plant_trace_value_7/1
  Torque/1 -> plant_trace_value_2/1
  Speed/1 -> plant_trace_value_1/1
  plant_trace_value_8/1 -> plant_trace_bus/8
  Id/1 -> plant_trace_value_3/1
  plant_trace_value_10/1 -> plant_trace_bus/10
  Iq/1 -> plant_trace_value_4/1
  plant_trace_bus/1 -> plant_trace/1
  plant_trace_value_9/1 -> plant_trace_bus/9
  plant_trace_value_3/1 -> plant_trace_bus/3
  plant_trace_value_2/1 -> plant_trace_bus/2
  plant_trace_value_4/1 -> plant_trace_bus/4
  Load/1 -> plant_trace_value_6/1
  plant_trace_value_7/1 -> plant_trace_bus/7
  plant_trace_value_6/1 -> plant_trace_bus/6
  plant_trace_value_1/1 -> plant_trace_bus/1
  plant_trace_value_5/1 -> plant_trace_bus/5

== system ChoiSul1996_DeadTime/IPMSM/Q_Axis_Electrical ==
  Vq : Inport
  OmegaE : Inport  Port=2
  Id : Inport  Port=3
  D_axis_speed_voltage : Product
  D_flux : Gain  Gain=Ld
  D_flux_total : Sum
  Delta_Iq : Gain  Gain=h/Lq
  Iq_state : UnitDelay  InitialCondition=double(0)  SampleTime=h  HasFrameUpgradeWarning=on
  Magnet_flux : Constant  Value=Psi  OutDataTypeStr=double
  Next_Iq : Sum
  Q_current_derivative : Sum  Inputs=+--
  Q_resistive_drop : Gain  Gain=R
  Iq : Outport
  wires:
  Vq/1 -> Q_current_derivative/1
  Id/1 -> D_flux/1
  D_flux_total/1 -> D_axis_speed_voltage/2
  Magnet_flux/1 -> D_flux_total/2
  D_flux/1 -> D_flux_total/1
  OmegaE/1 -> D_axis_speed_voltage/1
  Q_current_derivative/1 -> Delta_Iq/1
  D_axis_speed_voltage/1 -> Q_current_derivative/3
  Next_Iq/1 -> Iq_state/1
  Delta_Iq/1 -> Next_Iq/2
  Q_resistive_drop/1 -> Q_current_derivative/2
  Iq_state/1 -> Q_resistive_drop/1, Next_Iq/1, Iq/1

== system ChoiSul1996_DeadTime/IPMSM/Rotor_Angle ==
  OmegaE : Inport
  Angle_increment : Gain  Gain=h
  Electrical_angle : UnitDelay  InitialCondition=double(0)  SampleTime=h  HasFrameUpgradeWarning=on
  Next_angle : Sum
  Theta : Outport
  wires:
  OmegaE/1 -> Angle_increment/1
  Electrical_angle/1 -> Theta/1, Next_angle/1
  Next_angle/1 -> Electrical_angle/1
  Angle_increment/1 -> Next_angle/2

== system ChoiSul1996_DeadTime/IPMSM/Torque_And_Mechanics ==
  Load : Inport
  Iq : Inport  Port=2
  Id : Inport  Port=3
  Delta_speed : Gain  Gain=h/J
  Electrical_speed : Gain  Gain=Pairs
  Magnet_torque_flux : Constant  Value=Psi  OutDataTypeStr=double
  Mechanical_speed : UnitDelay  InitialCondition=double(0)  SampleTime=h  HasFrameUpgradeWarning=on
  Motor_torque : Gain  Gain=1.5*Pairs
  Net_torque : Sum  Inputs=+--
  Next_speed : Sum
  RPM : Gain  Gain=30/pi
  Reluctance_flux : Gain  Gain=Ld-Lq
  Torque_flux : Sum
  Torque_flux_times_current : Product
  Viscous_drag : Gain  Gain=B
  Speed : Outport
  Torque : Outport  Port=2
  OmegaE : Outport  Port=3
  wires:
  Id/1 -> Reluctance_flux/1
  Electrical_speed/1 -> OmegaE/1
  Load/1 -> Net_torque/2
  RPM/1 -> Speed/1
  Iq/1 -> Torque_flux_times_current/2
  Torque_flux_times_current/1 -> Motor_torque/1
  Torque_flux/1 -> Torque_flux_times_current/1
  Delta_speed/1 -> Next_speed/2
  Net_torque/1 -> Delta_speed/1
  Reluctance_flux/1 -> Torque_flux/2
  Mechanical_speed/1 -> Electrical_speed/1, Viscous_drag/1, Next_speed/1, RPM/1
  Magnet_torque_flux/1 -> Torque_flux/1
  Motor_torque/1 -> Net_torque/1, Torque/1
  Next_speed/1 -> Mechanical_speed/1
  Viscous_drag/1 -> Net_torque/3

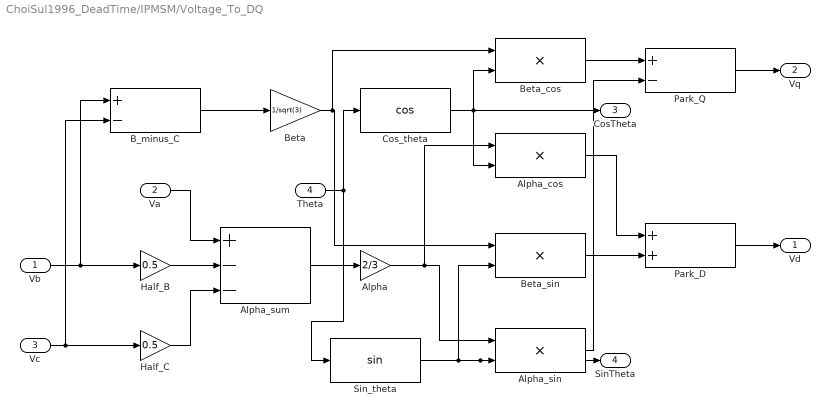
== system ChoiSul1996_DeadTime/IPMSM/Voltage_To_DQ ==
  Vb : Inport
  Va : Inport  Port=2
  Vc : Inport  Port=3
  Theta : Inport  Port=4
  Alpha : Gain  Gain=2/3
  Alpha_cos : Product
  Alpha_sin : Product
  Alpha_sum : Sum  Inputs=+--
  B_minus_C : Sum  Inputs=+-
  Beta : Gain  Gain=1/sqrt(3)
  Beta_cos : Product
  Beta_sin : Product
  Cos_theta : Trigonometry  Operator=cos
  Half_B : Gain  Gain=0.5
  Half_C : Gain  Gain=0.5
  Park_D : Sum
  Park_Q : Sum  Inputs=+-
  Sin_theta : Trigonometry
  Vd : Outport
  Vq : Outport  Port=2
  CosTheta : Outport  Port=3
  SinTheta : Outport  Port=4
  wires:
  Park_Q/1 -> Vq/1
  Vb/1 -> B_minus_C/1, Half_B/1
  Beta_cos/1 -> Park_Q/1
  Alpha_sum/1 -> Alpha/1
  Alpha_sin/1 -> Park_Q/2
  Beta_sin/1 -> Park_D/2
  Alpha_cos/1 -> Park_D/1
  Vc/1 -> B_minus_C/2, Half_C/1
  Sin_theta/1 -> SinTheta/1, Alpha_sin/2, Beta_sin/2
  Va/1 -> Alpha_sum/1
  Half_B/1 -> Alpha_sum/2
  Alpha/1 -> Alpha_sin/1, Alpha_cos/1
  Park_D/1 -> Vd/1
  Half_C/1 -> Alpha_sum/3
  Beta/1 -> Beta_cos/1, Beta_sin/1
  B_minus_C/1 -> Beta/1
  Cos_theta/1 -> Alpha_cos/2, Beta_cos/2, CosTheta/1
  Theta/1 -> Cos_theta/1, Sin_theta/1

== system ChoiSul1996_DeadTime/PWM_Inverter/PWM_Carrier ==
  Carrier_cycles : Gain  Gain=1/Ts
  Carrier_phase : Math  Operator=mod
  Centered_phase : Sum  Inputs=+-
  Half_cycle : Constant  Value=0.5  OutDataTypeStr=double
  Half_cycle_distance : Abs  SaturateOnIntegerOverflow=off
  One_cycle : Constant  OutDataTypeStr=double
  Plant_clock : DigitalClock  SampleTime=h
  Triangle : Gain  Gain=2
  Carrier : Outport
  wires:
  Triangle/1 -> Carrier/1
  Plant_clock/1 -> Carrier_cycles/1
  Carrier_cycles/1 -> Carrier_phase/1
  Centered_phase/1 -> Half_cycle_distance/1
  Carrier_phase/1 -> Centered_phase/1
  Half_cycle/1 -> Centered_phase/2
  One_cycle/1 -> Carrier_phase/2
  Half_cycle_distance/1 -> Triangle/1

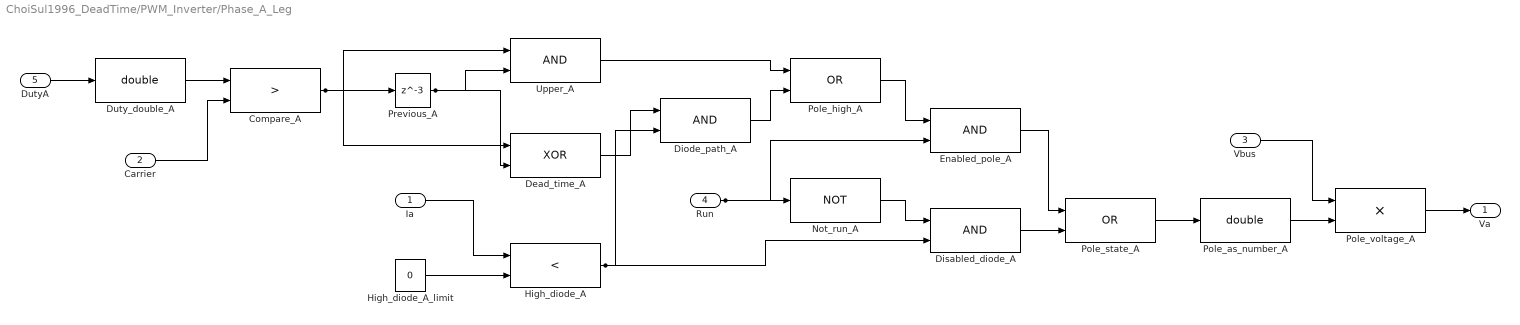
== system ChoiSul1996_DeadTime/PWM_Inverter/Phase_A_Leg ==
  Ia : Inport
  Carrier : Inport  Port=2
  Vbus : Inport  Port=3
  Run : Inport  Port=4
  DutyA : Inport  Port=5
  Compare_A : RelationalOperator  Operator=>  OutDataTypeStr=boolean  RndMeth=Simplest  InputSameDT=off
  Dead_time_A : Logic  Operator=XOR  IconShape=distinctive  AllPortsSameDT=off  OutDataTypeStr=boolean
  Diode_path_A : Logic  IconShape=distinctive  AllPortsSameDT=off  OutDataTypeStr=boolean
  Disabled_diode_A : Logic  IconShape=distinctive  AllPortsSameDT=off  OutDataTypeStr=boolean
  Duty_double_A : DataTypeConversion  OutDataTypeStr=double  SaturateOnIntegerOverflow=off  RndMeth=Floor
  Enabled_pole_A : Logic  IconShape=distinctive  AllPortsSameDT=off  OutDataTypeStr=boolean
  High_diode_A : RelationalOperator  Operator=<  OutDataTypeStr=boolean  RndMeth=Simplest  InputSameDT=off
  High_diode_A_limit : Constant  Value=0  OutDataTypeStr=double
  Not_run_A : Logic  Operator=NOT  Inputs=1  IconShape=distinctive  AllPortsSameDT=off  OutDataTypeStr=boolean
  Pole_as_number_A : DataTypeConversion  OutDataTypeStr=double  SaturateOnIntegerOverflow=off  RndMeth=Floor
  Pole_high_A : Logic  Operator=OR  IconShape=distinctive  AllPortsSameDT=off  OutDataTypeStr=boolean
  Pole_state_A : Logic  Operator=OR  IconShape=distinctive  AllPortsSameDT=off  OutDataTypeStr=boolean
  Pole_voltage_A : Product
  Previous_A : Delay  DelayLength=3  InitialCondition=0  SampleTime=h
  Upper_A : Logic  IconShape=distinctive  AllPortsSameDT=off  OutDataTypeStr=boolean
  Va : Outport
  wires:
  Ia/1 -> High_diode_A/1
  DutyA/1 -> Duty_double_A/1
  Pole_voltage_A/1 -> Va/1
  Vbus/1 -> Pole_voltage_A/1
  Carrier/1 -> Compare_A/2
  Pole_state_A/1 -> Pole_as_number_A/1
  Diode_path_A/1 -> Pole_high_A/2
  Duty_double_A/1 -> Compare_A/1
  High_diode_A_limit/1 -> High_diode_A/2
  Pole_high_A/1 -> Enabled_pole_A/1
  Not_run_A/1 -> Disabled_diode_A/1
  Run/1 -> Enabled_pole_A/2, Not_run_A/1
  High_diode_A/1 -> Diode_path_A/2, Disabled_diode_A/2
  Dead_time_A/1 -> Diode_path_A/1
  Pole_as_number_A/1 -> Pole_voltage_A/2
  Compare_A/1 -> Dead_time_A/1, Upper_A/1, Previous_A/1
  Upper_A/1 -> Pole_high_A/1
  Enabled_pole_A/1 -> Pole_state_A/1
  Disabled_diode_A/1 -> Pole_state_A/2
  Previous_A/1 -> Dead_time_A/2, Upper_A/2

== system ChoiSul1996_DeadTime/PWM_Inverter/Phase_B_Leg ==
  Carrier : Inport
  Vbus : Inport  Port=2
  Run : Inport  Port=3
  DutyB : Inport  Port=4
  Ib : Inport  Port=5
  Compare_B : RelationalOperator  Operator=>  OutDataTypeStr=boolean  RndMeth=Simplest  InputSameDT=off
  Dead_time_B : Logic  Operator=XOR  IconShape=distinctive  AllPortsSameDT=off  OutDataTypeStr=boolean
  Diode_path_B : Logic  IconShape=distinctive  AllPortsSameDT=off  OutDataTypeStr=boolean
  Disabled_diode_B : Logic  IconShape=distinctive  AllPortsSameDT=off  OutDataTypeStr=boolean
  Duty_double_B : DataTypeConversion  OutDataTypeStr=double  SaturateOnIntegerOverflow=off  RndMeth=Floor
  Enabled_pole_B : Logic  IconShape=distinctive  AllPortsSameDT=off  OutDataTypeStr=boolean
  High_diode_B : RelationalOperator  Operator=<  OutDataTypeStr=boolean  RndMeth=Simplest  InputSameDT=off
  High_diode_B_limit : Constant  Value=0  OutDataTypeStr=double
  Not_run_B : Logic  Operator=NOT  Inputs=1  IconShape=distinctive  AllPortsSameDT=off  OutDataTypeStr=boolean
  Pole_as_number_B : DataTypeConversion  OutDataTypeStr=double  SaturateOnIntegerOverflow=off  RndMeth=Floor
  Pole_high_B : Logic  Operator=OR  IconShape=distinctive  AllPortsSameDT=off  OutDataTypeStr=boolean
  Pole_state_B : Logic  Operator=OR  IconShape=distinctive  AllPortsSameDT=off  OutDataTypeStr=boolean
  Pole_voltage_B : Product
  Previous_B : Delay  DelayLength=3  InitialCondition=0  SampleTime=h
  Upper_B : Logic  IconShape=distinctive  AllPortsSameDT=off  OutDataTypeStr=boolean
  Vb : Outport
  wires:
  DutyB/1 -> Duty_double_B/1
  Vbus/1 -> Pole_voltage_B/1
  Diode_path_B/1 -> Pole_high_B/2
  Upper_B/1 -> Pole_high_B/1
  Enabled_pole_B/1 -> Pole_state_B/1
  Compare_B/1 -> Dead_time_B/1, Upper_B/1, Previous_B/1
  Not_run_B/1 -> Disabled_diode_B/1
  Carrier/1 -> Compare_B/2
  Ib/1 -> High_diode_B/1
  Pole_as_number_B/1 -> Pole_voltage_B/2
  High_diode_B/1 -> Diode_path_B/2, Disabled_diode_B/2
  Pole_high_B/1 -> Enabled_pole_B/1
  Pole_voltage_B/1 -> Vb/1
  Dead_time_B/1 -> Diode_path_B/1
  Disabled_diode_B/1 -> Pole_state_B/2
  High_diode_B_limit/1 -> High_diode_B/2
  Run/1 -> Not_run_B/1, Enabled_pole_B/2
  Duty_double_B/1 -> Compare_B/1
  Pole_state_B/1 -> Pole_as_number_B/1
  Previous_B/1 -> Dead_time_B/2, Upper_B/2

== system ChoiSul1996_DeadTime/PWM_Inverter/Phase_C_Leg ==
  Carrier : Inport
  Vbus : Inport  Port=2
  Ic : Inport  Port=3
  Run : Inport  Port=4
  DutyC : Inport  Port=5
  Compare_C : RelationalOperator  Operator=>  OutDataTypeStr=boolean  RndMeth=Simplest  InputSameDT=off
  Dead_time_C : Logic  Operator=XOR  IconShape=distinctive  AllPortsSameDT=off  OutDataTypeStr=boolean
  Diode_path_C : Logic  IconShape=distinctive  AllPortsSameDT=off  OutDataTypeStr=boolean
  Disabled_diode_C : Logic  IconShape=distinctive  AllPortsSameDT=off  OutDataTypeStr=boolean
  Duty_double_C : DataTypeConversion  OutDataTypeStr=double  SaturateOnIntegerOverflow=off  RndMeth=Floor
  Enabled_pole_C : Logic  IconShape=distinctive  AllPortsSameDT=off  OutDataTypeStr=boolean
  High_diode_C : RelationalOperator  Operator=<  OutDataTypeStr=boolean  RndMeth=Simplest  InputSameDT=off
  High_diode_C_limit : Constant  Value=0  OutDataTypeStr=double
  Not_run_C : Logic  Operator=NOT  Inputs=1  IconShape=distinctive  AllPortsSameDT=off  OutDataTypeStr=boolean
  Pole_as_number_C : DataTypeConversion  OutDataTypeStr=double  SaturateOnIntegerOverflow=off  RndMeth=Floor
  Pole_high_C : Logic  Operator=OR  IconShape=distinctive  AllPortsSameDT=off  OutDataTypeStr=boolean
  Pole_state_C : Logic  Operator=OR  IconShape=distinctive  AllPortsSameDT=off  OutDataTypeStr=boolean
  Pole_voltage_C : Product
  Previous_C : Delay  DelayLength=3  InitialCondition=0  SampleTime=h
  Upper_C : Logic  IconShape=distinctive  AllPortsSameDT=off  OutDataTypeStr=boolean
  Vc : Outport
  wires:
  Carrier/1 -> Compare_C/2
  Ic/1 -> High_diode_C/1
  Pole_voltage_C/1 -> Vc/1
  Diode_path_C/1 -> Pole_high_C/2
  Pole_state_C/1 -> Pole_as_number_C/1
  DutyC/1 -> Duty_double_C/1
  Pole_as_number_C/1 -> Pole_voltage_C/2
  Dead_time_C/1 -> Diode_path_C/1
  Duty_double_C/1 -> Compare_C/1
  Pole_high_C/1 -> Enabled_pole_C/1
  Compare_C/1 -> Upper_C/1, Dead_time_C/1, Previous_C/1
  Enabled_pole_C/1 -> Pole_state_C/1
  Upper_C/1 -> Pole_high_C/1
  High_diode_C/1 -> Diode_path_C/2, Disabled_diode_C/2
  Run/1 -> Not_run_C/1, Enabled_pole_C/2
  Disabled_diode_C/1 -> Pole_state_C/2
  Not_run_C/1 -> Disabled_diode_C/1
  Vbus/1 -> Pole_voltage_C/1
  High_diode_C_limit/1 -> High_diode_C/2
  Previous_C/1 -> Dead_time_C/2, Upper_C/2

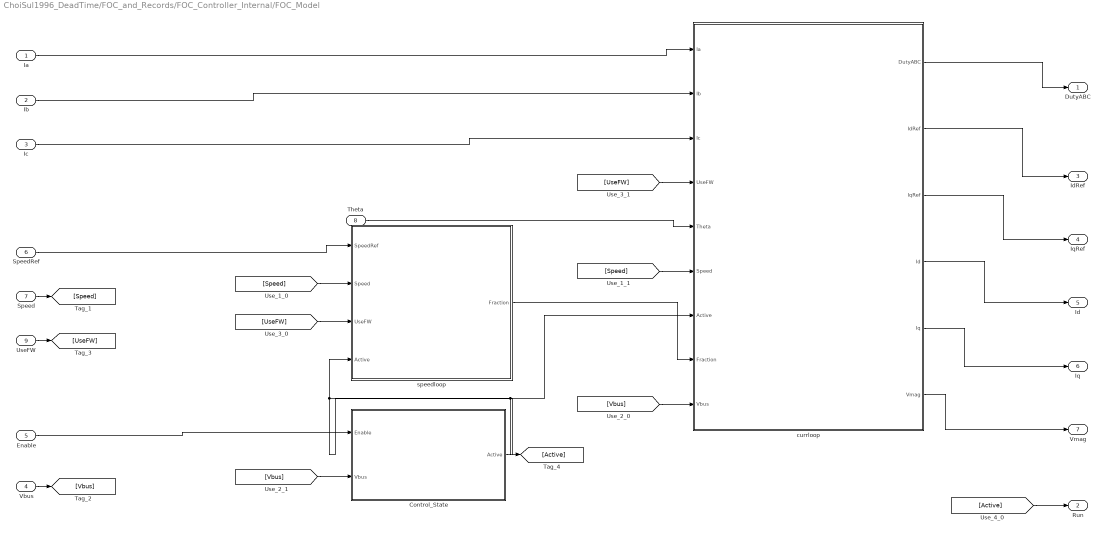
== system ChoiSul1996_DeadTime/FOC_and_Records/FOC_Controller_Internal/FOC_Model ==
  Ia : Inport
  Ib : Inport  Port=2
  Ic : Inport  Port=3
  Vbus : Inport  Port=4
  Enable : Inport  Port=5
  SpeedRef : Inport  Port=6
  Speed : Inport  Port=7
  Theta : Inport  Port=8
  UseFW : Inport  Port=9
  Control_State : Subsystem  TreatAsAtomicUnit=on
  currloop : Subsystem  TreatAsAtomicUnit=on
  speedloop : Subsystem  TreatAsAtomicUnit=on
  DutyABC : Outport
  Run : Outport  Port=2
  IdRef : Outport  Port=3
  IqRef : Outport  Port=4
  Id : Outport  Port=5
  Iq : Outport  Port=6
  Vmag : Outport  Port=7
  wires:
  currloop/6(Vmag) -> Vmag/1
  currloop/5(Iq) -> Iq/1
  currloop/4(Id) -> Id/1
  currloop/3(IqRef) -> IqRef/1
  currloop/2(IdRef) -> IdRef/1
  currloop/1(DutyABC) -> DutyABC/1
  Control_State/1(Active) -> speedloop/4(Active), currloop/7(Active), [Active]
  UseFW/1 -> [UseFW]
  Vbus/1 -> [Vbus]
  Speed/1 -> [Speed]
  [Speed] -> speedloop/2(Speed)
  [Speed] -> currloop/6(Speed)
  [Vbus] -> currloop/9(Vbus)
  [Vbus] -> Control_State/2(Vbus)
  [UseFW] -> speedloop/3(UseFW)
  [UseFW] -> currloop/4(UseFW)
  [Active] -> Run/1
  Ia/1 -> currloop/1(Ia)
  SpeedRef/1 -> speedloop/1(SpeedRef)
  Enable/1 -> Control_State/1(Enable)
  speedloop/1(Fraction) -> currloop/8(Fraction)
  Ic/1 -> currloop/3(Ic)
  Theta/1 -> currloop/5(Theta)
  Ib/1 -> currloop/2(Ib)

== system ChoiSul1996_DeadTime/FOC_and_Records/FOC_Controller_Internal/FOC_Model/Control_State ==
  Enable : Inport
  Vbus : Inport  Port=2
  Bus_ready : RelationalOperator  OutDataTypeStr=boolean  RndMeth=Simplest  InputSameDT=off
  Bus_ready_limit : Constant  Value=Vdc*BusReadyRatio  OutDataTypeStr=single
  Cmd_enabled : RelationalOperator  Operator=>  OutDataTypeStr=boolean  RndMeth=Simplest  InputSameDT=off
  Cmd_enabled_limit : Constant  Value=EnableThreshold  OutDataTypeStr=single
  Drive_enabled : Logic  IconShape=distinctive  AllPortsSameDT=off  OutDataTypeStr=boolean
  Active : Outport
  wires:
  Enable/1 -> Cmd_enabled/1
  Bus_ready/1 -> Drive_enabled/2
  Cmd_enabled_limit/1 -> Cmd_enabled/2
  Drive_enabled/1 -> Active/1
  Bus_ready_limit/1 -> Bus_ready/2
  Vbus/1 -> Bus_ready/1
  Cmd_enabled/1 -> Drive_enabled/1

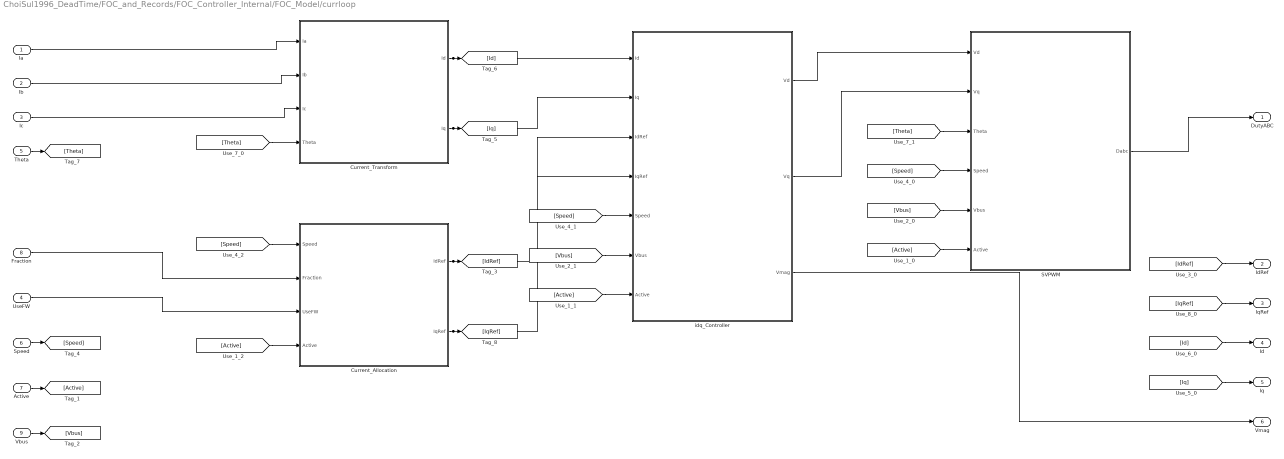
== system ChoiSul1996_DeadTime/FOC_and_Records/FOC_Controller_Internal/FOC_Model/currloop ==
  Ia : Inport
  Ib : Inport  Port=2
  Ic : Inport  Port=3
  UseFW : Inport  Port=4
  Theta : Inport  Port=5
  Speed : Inport  Port=6
  Active : Inport  Port=7
  Fraction : Inport  Port=8
  Vbus : Inport  Port=9
  Current_Allocation : Subsystem  TreatAsAtomicUnit=on
  Current_Transform : Subsystem  TreatAsAtomicUnit=on
  SVPWM : Subsystem  TreatAsAtomicUnit=on
  idq_Controller : Subsystem  TreatAsAtomicUnit=on
  DutyABC : Outport
  IdRef : Outport  Port=2
  IqRef : Outport  Port=3
  Id : Outport  Port=4
  Iq : Outport  Port=5
  Vmag : Outport  Port=6
  wires:
  Current_Allocation/2(IqRef) -> [IqRef], idq_Controller/4(IqRef)
  Theta/1 -> [Theta]
  idq_Controller/2(Vq) -> SVPWM/2(Vq)
  Ib/1 -> Current_Transform/2(Ib)
  Current_Transform/1(Id) -> [Id], idq_Controller/1(Id)
  Current_Transform/2(Iq) -> idq_Controller/2(Iq), [Iq]
  Speed/1 -> [Speed]
  idq_Controller/1(Vd) -> SVPWM/1(Vd)
  Ic/1 -> Current_Transform/3(Ic)
  Current_Allocation/1(IdRef) -> [IdRef], idq_Controller/3(IdRef)
  Vbus/1 -> [Vbus]
  UseFW/1 -> Current_Allocation/3(UseFW)
  idq_Controller/3(Vmag) -> Vmag/1
  Fraction/1 -> Current_Allocation/2(Fraction)
  Ia/1 -> Current_Transform/1(Ia)
  SVPWM/1(Dabc) -> DutyABC/1
  Active/1 -> [Active]
  [Active] -> SVPWM/6(Active)
  [Active] -> idq_Controller/7(Active)
  [Active] -> Current_Allocation/4(Active)
  [Vbus] -> SVPWM/5(Vbus)
  [Vbus] -> idq_Controller/6(Vbus)
  [IdRef] -> IdRef/1
  [Speed] -> SVPWM/4(Speed)
  [Speed] -> idq_Controller/5(Speed)
  [Speed] -> Current_Allocation/1(Speed)
  [Iq] -> Iq/1
  [Id] -> Id/1
  [Theta] -> Current_Transform/4(Theta)
  [Theta] -> SVPWM/3(Theta)
  [IqRef] -> IqRef/1

== system ChoiSul1996_DeadTime/FOC_and_Records/FOC_Controller_Internal/FOC_Model/speedloop ==
  SpeedRef : Inport
  Speed : Inport  Port=2
  UseFW : Inport  Port=3
  Active : Inport  Port=4
  Speed_PI : Subsystem
  Torque_Capacity : Subsystem
  Torque_Normalization : Subsystem
  Fraction : Outport
  wires:
  Speed/1 -> [Speed]
  [Speed] -> Speed_PI/4(Speed)
  [Speed] -> Torque_Capacity/2(Speed)
  Torque_Normalization/1(Fraction) -> Fraction/1
  Speed_PI/1(TorqueCmd) -> Torque_Normalization/1(TorqueCmd)
  Active/1 -> Speed_PI/2(Active)
  SpeedRef/1 -> Speed_PI/1(SpeedRef)
  UseFW/1 -> Torque_Capacity/1(UseFW)
  Torque_Capacity/1(TorqueCap) -> Torque_Normalization/2(TorqueCap), Speed_PI/3(TorqueCap)

== system ChoiSul1996_DeadTime/FOC_and_Records/FOC_Controller_Internal/FOC_Model/currloop/Current_Allocation ==
  Speed : Inport
  Fraction : Inport  Port=2
  UseFW : Inport  Port=3
  Active : Inport  Port=4
  Enabled_IdRef : Product
  Enabled_IqRef : Product
  FW_d_map : Lookup_n-D  BreakpointsForDimension1=Ngrid  BreakpointsForDimension2=Fraction  BreakpointsForDimension3=[5, 7]  Table=FwId  ExtrapMethod=Clip  InternalRulePriority=Speed  RndMeth=Simplest
      settings: InputPortMap=u0,u1
  FW_q_map : Lookup_n-D  BreakpointsForDimension1=Ngrid  BreakpointsForDimension2=Fraction  BreakpointsForDimension3=[5, 7]  Table=FwIq  ExtrapMethod=Clip  InternalRulePriority=Speed  RndMeth=Simplest
      settings: InputPortMap=u0,u1
  MTPA_d_map : Lookup_n-D  BreakpointsForDimension1=Ngrid  BreakpointsForDimension2=Fraction  BreakpointsForDimension3=[5, 7]  Table=BaseId  ExtrapMethod=Clip  InternalRulePriority=Speed  RndMeth=Simplest
      settings: InputPortMap=u0,u1
  MTPA_q_map : Lookup_n-D  BreakpointsForDimension1=Ngrid  BreakpointsForDimension2=Fraction  BreakpointsForDimension3=[5, 7]  Table=BaseIq  ExtrapMethod=Clip  InternalRulePriority=Speed  RndMeth=Simplest
      settings: InputPortMap=u0,u1
  Select_d : Switch  Criteria=u2 > Threshold  Threshold=0.5  SaturateOnIntegerOverflow=off  InputSameDT=off
  Select_q : Switch  Criteria=u2 > Threshold  Threshold=0.5  SaturateOnIntegerOverflow=off  InputSameDT=off
  Speed_magnitude : Abs  SaturateOnIntegerOverflow=off
  IdRef : Outport
  IqRef : Outport  Port=2
  wires:
  Enabled_IqRef/1 -> IqRef/1
  Enabled_IdRef/1 -> IdRef/1
  Active/1 -> Enabled_IqRef/2, Enabled_IdRef/2
  Select_q/1 -> Enabled_IqRef/1
  Select_d/1 -> Enabled_IdRef/1
  MTPA_d_map/1 -> Select_d/3
  MTPA_q_map/1 -> Select_q/3
  FW_q_map/1 -> Select_q/1
  FW_d_map/1 -> Select_d/1
  Fraction/1 -> MTPA_q_map/2, FW_q_map/2, FW_d_map/2, MTPA_d_map/2
  Speed_magnitude/1 -> FW_q_map/1, MTPA_q_map/1, FW_d_map/1, MTPA_d_map/1
  Speed/1 -> Speed_magnitude/1
  UseFW/1 -> Select_q/2, Select_d/2

== system ChoiSul1996_DeadTime/FOC_and_Records/FOC_Controller_Internal/FOC_Model/currloop/Current_Transform ==
  Ia : Inport
  Ib : Inport  Port=2
  Ic : Inport  Port=3
  Theta : Inport  Port=4
  Clarke : Subsystem
  Park : Subsystem
  SinCos : Subsystem
  Id : Outport
  Iq : Outport  Port=2
  wires:
  SinCos/2(SinTheta) -> Park/4(SinTheta)
  SinCos/1(CosTheta) -> Park/3(CosTheta)
  Theta/1 -> SinCos/1(Theta)
  Park/2(Id) -> Id/1
  Park/1(Iq) -> Iq/1
  Clarke/2(Ibeta) -> Park/2(Ibeta)
  Clarke/1(Ialpha) -> Park/1(Ialpha)
  Ic/1 -> Clarke/3(Ic)
  Ib/1 -> Clarke/2(Ib)
  Ia/1 -> Clarke/1(Ia)
